simulink model "parametri_kp_ki_kd"  (R2015b)
settings: Solver=FixedStepAuto  StartTime=0.0  StopTime=20  RelTol=1e-3
libraries: simulink x1
settings Model: Creator=pc  LastModifiedBy=Elma

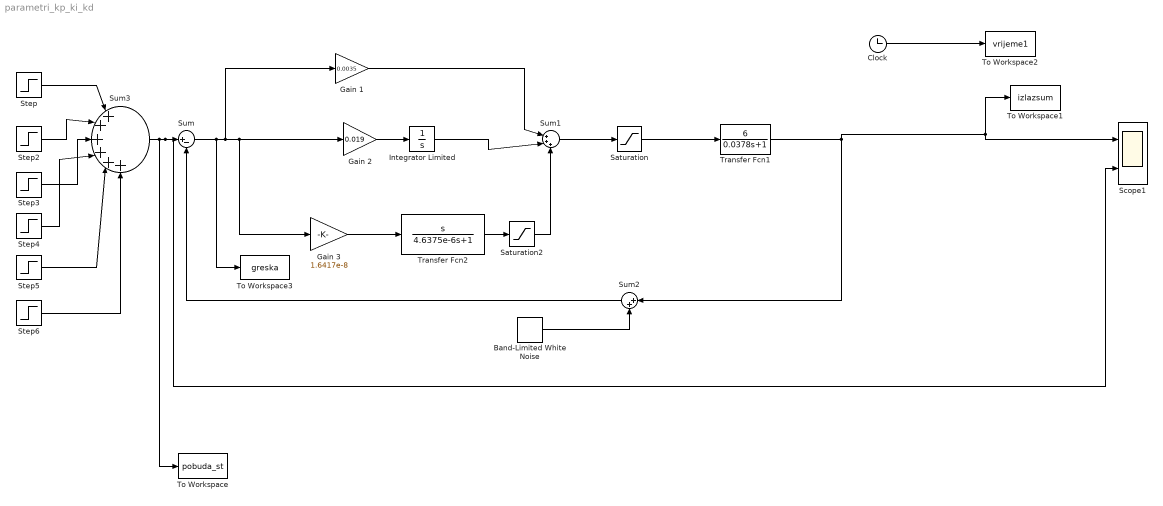
== system parametri_kp_ki_kd ==
  Band-Limited White Noise : simulink/Sources/Band-Limited White Noise  Cov=[0.1]  Ts=0.1  seed=[23341]
  Clock : Clock
  Gain 1 : Gain  Gain=0.0035
  Gain 2 : Gain  Gain=0.019
  Gain 3 : Gain  Gain=1.6417e-8
  Integrator Limited : Integrator  LimitOutput=on  UpperSaturationLimit=10  LowerSaturationLimit=0
  Saturation : Saturate  UpperLimit=10  LowerLimit=0
  Saturation2 : Saturate  UpperLimit=5  LowerLimit=0
  Scope1 : Scope  NumInputPorts=2
  Step : Step  After=60  SampleTime=0
  Step2 : Step  Time=4  After=-10  SampleTime=0
  Step3 : Step  Time=10  After=-25  SampleTime=0
  Step4 : Step  Time=12  After=14  SampleTime=0
  Step5 : Step  Time=14  After=6  SampleTime=0
  Step6 : Step  Time=20  After=-40  SampleTime=0
  Sum : Sum  Inputs=|+-
  Sum1 : Sum  Inputs=|+++
  Sum2 : Sum  Inputs=|++
  Sum3 : Sum  Inputs=|++++++
  To Workspace : ToWorkspace  VariableName=pobuda_st  SampleTime=-1
      settings: Save2DSignal=2-D array (concatenate along first dimension)
  To Workspace1 : ToWorkspace  VariableName=izlazsum  SampleTime=-1
      settings: Save2DSignal=2-D array (concatenate along first dimension)
  To Workspace2 : ToWorkspace  VariableName=vrijeme1  SampleTime=-1
      settings: Save2DSignal=2-D array (concatenate along first dimension)
  To Workspace3 : ToWorkspace  VariableName=greska  SampleTime=-1
      settings: Save2DSignal=2-D array (concatenate along first dimension)
  Transfer Fcn1 : TransferFcn  Numerator=[6]  Denominator=[0.0378 1]
  Transfer Fcn2 : TransferFcn  Numerator=[ 1 0 ]  Denominator=[4.6375e-6 1]
  wires:
  Sum3/1 -> Scope1/2, Sum/1, To Workspace/1
  Sum/1 -> Gain 3/1, Gain 2/1, Gain 1/1, To Workspace3/1
  Gain 1/1 -> Sum1/1
  Saturation/1 -> Transfer Fcn1/1
  Transfer Fcn1/1 -> Scope1/1, To Workspace1/1, Sum2/1
  Gain 2/1 -> Integrator Limited/1
  Clock/1 -> To Workspace2/1
  Band-Limited White Noise/1 -> Sum2/2
  Gain 3/1 -> Transfer Fcn2/1
  Integrator Limited/1 -> Sum1/2
  Sum1/1 -> Saturation/1
  Transfer Fcn2/1 -> Saturation2/1
  Sum2/1 -> Sum/2
  Step/1 -> Sum3/1
  Step2/1 -> Sum3/2
  Step3/1 -> Sum3/3
  Step4/1 -> Sum3/4
  Step5/1 -> Sum3/5
  Step6/1 -> Sum3/6
  Saturation2/1 -> Sum1/3
